simulink model "fi_pm"  (R2026a)
settings: Solver=FixedStepAuto  StopTime=50  FixedStep=1e-3  EnableMultiTasking=on
settings Model: PacingRate=0.250000  ExtModeTrigDuration=5  Creator=Arun Mistry  LastModifiedBy=harry_31916
settings OptimizationCC: DefaultUnderspecifiedDataType=single
settings HardwareCC: ProdLargestAtomicInteger=Long  ProdLargestAtomicFloat=Double  ProdHWDeviceType=ARM Compatible->ARM Cortex
settings SFSimCC: SimParseCustomCode=off
settings RTWCC: SystemTargetFile=ert.tlc  Toolchain=GNU Tools for ARM Embedded Processors  Description=Embedded Coder
settings ERTTargetCC: DynamicArrayContainerType=coder::array

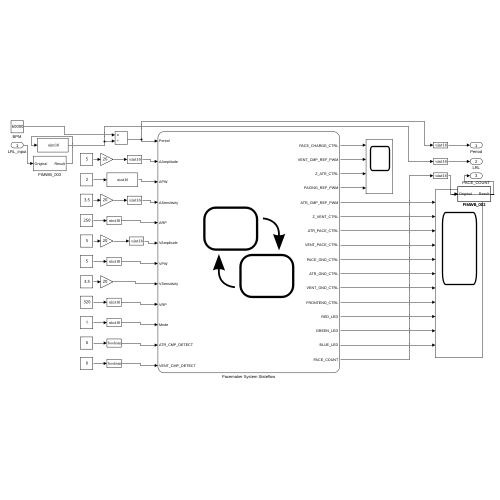
[thumbnail: Simulink's stored preview of the top-level diagram]
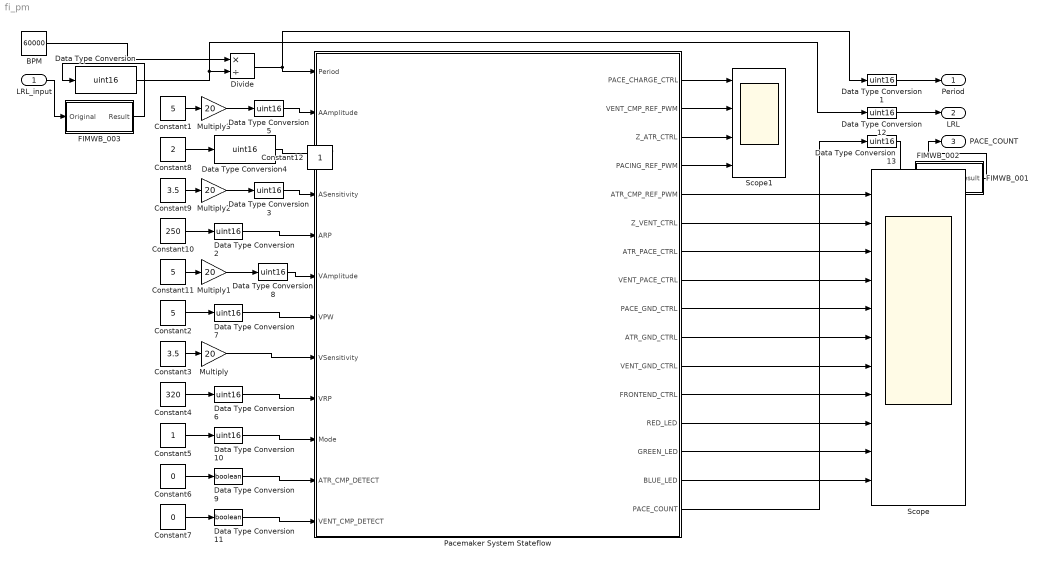
== system fi_pm ==
  LRL_input : Inport  OutDataTypeStr=double
  BPM : Constant  Value=60000
  Constant1 : Constant  Value=5
  Constant10 : Constant  Value=250
  Constant11 : Constant  Value=5
  Constant2 : Constant  Value=5
  Constant3 : Constant  Value=3.5
  Constant4 : Constant  Value=320
  Constant5 : Constant
  Constant6 : Constant  Value=0
  Constant7 : Constant  Value=0
  Constant8 : Constant  Value=2
  Constant9 : Constant  Value=3.5
  Data Type Conversion{,1..8,10,12..13} (12 alike) : DataTypeConversion  OutDataTypeStr=uint16  SaturateOnIntegerOverflow=off  RndMeth=Floor
  Data Type Conversion11 : DataTypeConversion  OutDataTypeStr=boolean  SaturateOnIntegerOverflow=off  RndMeth=Floor
  Data Type Conversion9 : DataTypeConversion  OutDataTypeStr=boolean  SaturateOnIntegerOverflow=off  RndMeth=Floor
  Divide : Product  Inputs=*/
  FIMWB_001 : Subsystem  Tag=fimwb.fault.1
  FIMWB_002 : Subsystem  Tag=fimwb.fault.2
  FIMWB_003 : Subsystem  Tag=fimwb.fault.3
  Multiply{,1..3} (4 alike) : Gain  Gain=20
  Pacemaker System Stateflow : Stateflow chart  TreatAsAtomicUnit=on
  Scope : Scope  NumInputPorts=11
  Scope1 : Scope  NumInputPorts=4
  Period : Outport  OutDataTypeStr=uint16
  LRL : Outport  Port=2  OutDataTypeStr=uint16
  PACE_COUNT : Outport  Port=3
  Constant12 : Constant  IOType=siggen
  wires:
  Constant2/1 -> Data Type Conversion7/1
  Constant7/1 -> Data Type Conversion11/1
  Constant8/1 -> Data Type Conversion4/1
  Pacemaker System Stateflow/7(ATR_PACE_CTRL) -> Scope/3
  Pacemaker System Stateflow/10(ATR_GND_CTRL) -> Scope/6
  Constant5/1 -> Data Type Conversion10/1
  Pacemaker System Stateflow/6(Z_VENT_CTRL) -> Scope/2
  Pacemaker System Stateflow/11(VENT_GND_CTRL) -> Scope/7
  Pacemaker System Stateflow/9(PACE_GND_CTRL) -> Scope/5
  Pacemaker System Stateflow/8(VENT_PACE_CTRL) -> Scope/4
  Pacemaker System Stateflow/15(BLUE_LED) -> Scope/11
  Pacemaker System Stateflow/12(FRONTEND_CTRL) -> Scope/8
  Constant10/1 -> Data Type Conversion2/1
  Pacemaker System Stateflow/14(GREEN_LED) -> Scope/10
  Pacemaker System Stateflow/13(RED_LED) -> Scope/9
  Pacemaker System Stateflow/5(ATR_CMP_REF_PWM) -> Scope/1
  Multiply1/1 -> Data Type Conversion8/1
  Multiply2/1 -> Data Type Conversion3/1
  Multiply3/1 -> Data Type Conversion5/1
  BPM/1 -> Divide/1
  Divide/1 -> Data Type Conversion1/1, Pacemaker System Stateflow/1(Period)
  Pacemaker System Stateflow/1(PACE_CHARGE_CTRL) -> Scope1/1
  Pacemaker System Stateflow/2(VENT_CMP_REF_PWM) -> Scope1/2
  Pacemaker System Stateflow/3(Z_ATR_CTRL) -> Scope1/3
  Pacemaker System Stateflow/4(PACING_REF_PWM) -> Scope1/4
  Data Type Conversion/1 -> Data Type Conversion12/1, Divide/2
  Data Type Conversion1/1 -> Period/1
  Constant1/1 -> Multiply3/1
  Data Type Conversion4/1 -> Pacemaker System Stateflow/3(APW)
  Constant9/1 -> Multiply2/1
  Data Type Conversion2/1 -> Pacemaker System Stateflow/5(ARP)
  Constant6/1 -> Data Type Conversion9/1
  Data Type Conversion10/1 -> Pacemaker System Stateflow/10(Mode)
  Constant4/1 -> Data Type Conversion6/1
  Constant11/1 -> Multiply1/1
  Data Type Conversion7/1 -> Pacemaker System Stateflow/7(VPW)
  Data Type Conversion5/1 -> Pacemaker System Stateflow/2(AAmplitude)
  Data Type Conversion3/1 -> Pacemaker System Stateflow/4(ASensitivity)
  Data Type Conversion8/1 -> Pacemaker System Stateflow/6(VAmplitude)
  Constant3/1 -> Multiply/1
  Multiply/1 -> Pacemaker System Stateflow/8(VSensitivity)
  Data Type Conversion6/1 -> Pacemaker System Stateflow/9(VRP)
  Data Type Conversion11/1 -> Pacemaker System Stateflow/12(VENT_CMP_DETECT)
  Data Type Conversion9/1 -> Pacemaker System Stateflow/11(ATR_CMP_DETECT)
  Pacemaker System Stateflow/16(PACE_COUNT) -> Data Type Conversion13/1
  Data Type Conversion12/1 -> LRL/1
  Data Type Conversion13/1 -> FIMWB_001/1(Original)
  FIMWB_001/1(Result) -> FIMWB_002/1(Original)
  FIMWB_002/1(Result) -> PACE_COUNT/1
  LRL_input/1 -> FIMWB_003/1(Original)
  FIMWB_003/1(Result) -> Data Type Conversion/1

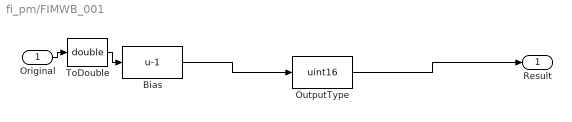
== system fi_pm/FIMWB_001 ==
  Original : Inport
  Bias : Bias  Bias=-1  SaturateOnIntegerOverflow=off
  OutputType : DataTypeConversion  OutDataTypeStr=uint16  RndMeth=Round
  ToDouble : DataTypeConversion  OutDataTypeStr=double  SaturateOnIntegerOverflow=off  RndMeth=Floor
  Result : Outport
  wires:
  Original/1 -> ToDouble/1
  ToDouble/1 -> Bias/1
  Bias/1 -> OutputType/1
  OutputType/1 -> Result/1

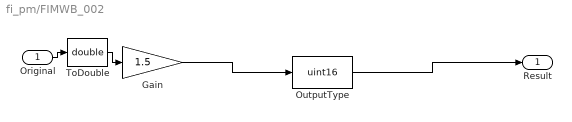
== system fi_pm/FIMWB_002 ==
  Original : Inport
  Gain : Gain  Gain=1.5  OutDataTypeStr=Inherit: Same as input
  OutputType : DataTypeConversion  OutDataTypeStr=uint16  RndMeth=Round
  ToDouble : DataTypeConversion  OutDataTypeStr=double  SaturateOnIntegerOverflow=off  RndMeth=Floor
  Result : Outport
  wires:
  Original/1 -> ToDouble/1
  ToDouble/1 -> Gain/1
  Gain/1 -> OutputType/1
  OutputType/1 -> Result/1

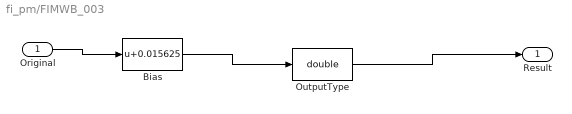
== system fi_pm/FIMWB_003 ==
  Original : Inport
  Bias : Bias  Bias=0.015625  SaturateOnIntegerOverflow=off
  OutputType : DataTypeConversion  OutDataTypeStr=double  RndMeth=Round
  Result : Outport
  wires:
  Original/1 -> Bias/1
  Bias/1 -> OutputType/1
  OutputType/1 -> Result/1

== stateflow chart fi_pm/Pacemaker System Stateflow ==
  state AOO
    entry: % Initialize pin assigments that do not change during the states
    VENT_PACE_CTRL = 0; VENT_GND_CTRL = 0; PACE_GND_CTRL = 1;
    Z_VENT_CTRL = 0; Z_ATR_CTRL = 0;
    PACING_REF_PWM = AAmplitude; PACE_COUNT = 0;
    state PACE_ATR
      entry:
      % STOP CHARGING C22
      PACE_CHARGE_CTRL = 0;
      % DISCHARGE C22 THROUGH ATR
      ATR_GND_CTRL = 0;
      ATR_PACE_CTRL = 1;
      % PULSING INDICATOR
      BLUE_LED = 1;
      PACE_COUNT = PACE_COUNT + 1;
    state CHARGE_CAPACITOR
      entry:
      % DISCONNECT ATRIAL PACING
      ATR_PACE_CTRL = 0;
      % DISCONNECT C21 FROM GND (allow charge buildup)
      ATR_GND_CTRL = 1;
      % CHARGING C22
      PACE_CHARGE_CTRL = 1;
      % DISABLE PULSING INDICATOR
      BLUE_LED = 0;
    (default) -> AOO.CHARGE_CAPACITOR
    AOO.PACE_ATR -> AOO.CHARGE_CAPACITOR : after(APW,msec)
    AOO.CHARGE_CAPACITOR -> AOO.PACE_ATR : after(Period - 70*APW,msec)
  state MODE_ROUTER
    entry: % Reset these pins when swithching between states
    FRONTEND_CTRL = 1;
    ATR_PACE_CTRL = 0;
    ATR_GND_CTRL = 0;
    VENT_GND_CTRL = 0;
    VENT_PACE_CTRL = 0;
    Z_ATR_CTRL = 0;
    Z_VENT_CTRL = 0;
    GREEN_LED = 0;
    RED_LED = 0;
    BLUE_LED = 0;
  state VOO
    entry: % Initialize pin assigments that do not change during the states
    ATR_PACE_CTRL = 0; ATR_GND_CTRL = 0; PACE_GND_CTRL = 1;
    Z_ATR_CTRL = 0; Z_VENT_CTRL = 0; PACING_REF_PWM = VAmplitude;
    state PACE_VENT
      entry:
      % STOP CHARGING C22
      PACE_CHARGE_CTRL = 0;
      % DISCHARGE C22 THROUGH VENT
      VENT_GND_CTRL = 0;
      VENT_PACE_CTRL = 1;
      % PULSING INDICATOR
      BLUE_LED = 1;
    state CHARGE_CAPACITOR
      entry:
      % DISCONNECT VENT PACING
      VENT_PACE_CTRL = 0;
      % DISCONNECT C21 FROM GND (allow charge to buildup)
      VENT_GND_CTRL = 1;
      % CHARGING C22
      PACE_CHARGE_CTRL = 1;
      % DISABLE PULSING INDICATOR
      BLUE_LED = 0;
    (default) -> VOO.CHARGE_CAPACITOR
    VOO.PACE_VENT -> VOO.CHARGE_CAPACITOR : after(VPW,msec)
    VOO.CHARGE_CAPACITOR -> VOO.PACE_VENT : after(Period-VPW,msec)
  state AAI
    % Initialize pin assignments that do not change during the states
    entry: VENT_PACE_CTRL = 0; VENT_GND_CTRL = 0; PACE_GND_CTRL = 1;
    Z_VENT_CTRL = 0; Z_ATR_CTRL = 0; FRONTEND_CTRL = 1;
    PACING_REF_PWM = AAmplitude; ATR_CMP_REF_PWM=ASensitivity;
    state PACE_ATR
      entry:
      % STOP CHARGING C22
      PACE_CHARGE_CTRL = 0;
      % DISCHARGE C22 THROUGH ATR
      ATR_PACE_CTRL = 1;
      ATR_GND_CTRL = 0;
      % PULSING INDICATOR
      BLUE_LED = 1;
    state C22_CHARGE
      entry:
      % DISCONNECT VENT PACING
      ATR_PACE_CTRL = 0;
      % DISCONNECT C21 FROM GND (allow charge to buildup)
      ATR_GND_CTRL = 1;
      % CHARGING C22
      PACE_CHARGE_CTRL = 1;
    state REFRACTORY_STATE
      % DISABLE PULSING INDICATORS
      entry: BLUE_LED = 0; PACE_CHARGE_CTRL = 1;
      ATR_PACE_CTRL = 0;  ATR_GND_CTRL = 1;
      % DISABLE INHIBIT INIDCATOR ON EXIT
      exit: GREEN_LED = 0;
    (default) -> C22_CHARGE
    C22_CHARGE -> AAI.PACE_ATR [order 2] : after(Period - ARP, msec)
    C22_CHARGE -> REFRACTORY_STATE [order 1] : [ATR_CMP_DETECT]
        | {GREEN_LED = 1}
    REFRACTORY_STATE -> C22_CHARGE : after(ARP, msec)
    AAI.PACE_ATR -> REFRACTORY_STATE : after(APW, msec)
  state VVI
    % Initialize pin assignments that do not change during the states
    entry: ATR_PACE_CTRL = 0; ATR_GND_CTRL = 0; PACE_GND_CTRL = 1;
    Z_VENT_CTRL = 0; Z_ATR_CTRL = 0; FRONTEND_CTRL = 1;
    PACING_REF_PWM = VAmplitude; VENT_CMP_REF_PWM = VSensitivity;
    state PACE_VENT
      entry:
      % STOP CHARGING C22
      PACE_CHARGE_CTRL = 0;
      % DISCHARGE C22 THROUGH VENT
      VENT_PACE_CTRL = 1;
      VENT_GND_CTRL = 0;
      % PULSING INDICATOR
      BLUE_LED = 1;
    state CHARGE_CAPACITOR
      entry:
      % CHARGING C22
      PACE_CHARGE_CTRL = 1;
      % DISCONNECT VENT PACING
      VENT_PACE_CTRL = 0;
      % DISCONNECT FROM GND
      VENT_GND_CTRL = 1;
    state REFRACTORY
      % DISABLE PULSING INDICATOR
      entry: BLUE_LED = 0; PACE_CHARGE_CTRL = 1;
      VENT_PACE_CTRL = 0;  VENT_GND_CTRL = 1;
      % DISABLE INHIBIT INDICATOR ON EXIT (if on)
      exit: GREEN_LED = 0;
    (default) -> VVI.CHARGE_CAPACITOR
    VVI.CHARGE_CAPACITOR -> VVI.PACE_VENT [order 2] : after(Period - VRP, msec)
    VVI.CHARGE_CAPACITOR -> REFRACTORY [order 1] : [VENT_CMP_DETECT]
        | {GREEN_LED = 1}
    REFRACTORY -> VVI.CHARGE_CAPACITOR : after(VRP, msec)
    VVI.PACE_VENT -> REFRACTORY : after(VPW, msec)
  (default) -> MODE_ROUTER
  MODE_ROUTER -> VOO [order 2] : [Mode==2]
  MODE_ROUTER -> AOO [order 1] : [Mode==1]
  VOO -> MODE_ROUTER : [Mode~=2]
  AOO -> MODE_ROUTER : [Mode~=1]
  MODE_ROUTER -> AAI [order 3] : [Mode==3]
  MODE_ROUTER -> VVI [order 4] : [Mode==4]
  AAI -> MODE_ROUTER : [Mode~=3]
  VVI -> MODE_ROUTER : [Mode~=4]
  data: Period input double; AAmplitude input uint16; APW input uint16; ASensitivity input uint16; ARP input uint16; VAmplitude input uint16; VPW input uint16; VSensitivity input double; VRP input uint16; PACE_CHARGE_CTRL output double; VENT_CMP_REF_PWM output double; Z_ATR_CTRL output double; PACING_REF_PWM output uint16; ATR_CMP_REF_PWM output uint16; Z_VENT_CTRL output uint16; ATR_PACE_CTRL output uint16; VENT_PACE_CTRL output uint16; PACE_GND_CTRL output uint16; ATR_GND_CTRL output uint16; VENT_GND_CTRL output uint16; Mode input uint16; FRONTEND_CTRL output uint16; RED_LED output uint16; GREEN_LED output uint16; BLUE_LED output uint16; ATR_CMP_DETECT input boolean; VENT_CMP_DETECT input boolean; PACE_COUNT output
